simulink model "emso3"  (Simulink 7.1)
settings: Solver=VariableStepDiscrete  StartTime=0.0  StopTime=360  RelTol=1e-3
settings Model: Creator=lades  LastModifiedBy=lades
settings DataIOCC: ExternalInput=Az

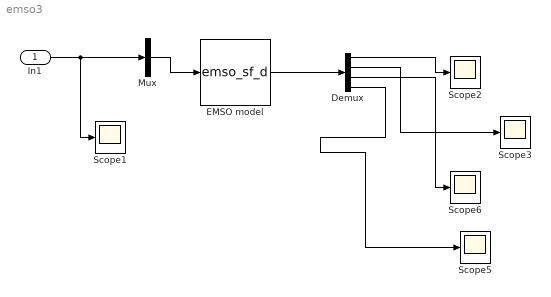
== system emso3 ==
  In1 : Inport  OutDataType=sfix(16)  OutScaling=2^0
  Demux : Demux
  EMSO model : S-Function  FunctionName=emso_sf_d  Parameters='batch_PID.ems',1,4,0.1  EnableBusSupport=off
  Mux : Mux  Inputs=1
  Scope{1..3,5..6} (5 alike) : Scope
      Scope1 settings: TimeRange=2  YMin=4.008258966500001  YMax=4.008258969500001
      Scope2 settings: TimeRange=2  YMin=0.750378  YMax=0.829366  SaveName=ScopeData2
      Scope3 settings: TimeRange=2  YMin=0.750378  YMax=0.829366
      Scope5 settings: TimeRange=2  YMin=0.750378  YMax=0.829366  SaveName=ScopeData4
      Scope6 settings: TimeRange=2  YMin=0.750378  YMax=0.829366  SaveName=ScopeData5
  wires:
  EMSO model/1 -> Demux/1
  Mux/1 -> EMSO model/1
  Demux/1 -> Scope2/1
  In1/1 -> Mux/1, Scope1/1
  Demux/4 -> Scope5/1
  Demux/3 -> Scope6/1
  Demux/2 -> Scope3/1
